simulink library "lib_AC_GFM"  (R2026a)
settings: Solver=VariableStepAuto
undefined symbols (not defined in the file): block_buses, block_idx, block_toM, buses_lf, fref, iC, invL, iR, iTf, op_GFM
libraries: simulink x4
(part 1 of 2)
settings Model: Creator=atomas  LastModifiedBy=atomas

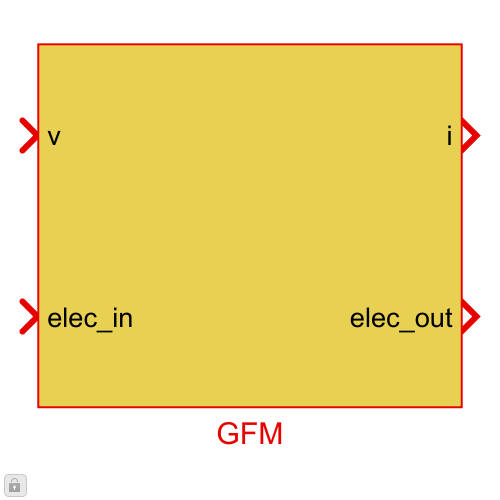
[thumbnail: Simulink's stored preview of the top-level diagram]
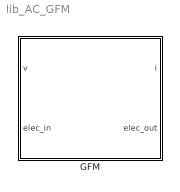
== system lib_AC_GFM ==
  GFM : Subsystem  mask(GFr){Pmax=Inf, Qmax=Inf, fb=50, dynamic_VCC=Static, Lf=0.01, Rf=0.001, Rcf=1000000, Cfi=0.1, Kint=1, Tint=0.1, Bint=1, Kext=1, Bext=1, Text=0.1, Fi=1, Tf=0.01, mp=0.01, mD=0, nq=0.01, VI_L=0.1, VI_R=0.01, WOF_Tf=0, L_out=0.1, R_out=0.01}
      mask prompts: Pmax "Active power limit (p.u.)"; Qmax "Reactive power limit (p.u.)"; fb "Base frequency (Hz)"; dynamic_VCC "Dynamic behavior"; Lf "Filter inductance (pu)"; Rf "Filter resistance (pu)"; Rcf "Parallel resistance to C (pu)"; Cfi "Filter capacitance (pu)"; Fi "Current feedfordward gain"; Tf "Low-pass filter time constant (s)"; mp "Droop coefficient mp (pu)"; mD "Droop coefficient mD (pu)"; nq "Droop coefficient nq (pu)"; VI_L "Inductance (pu)"; VI_R "Resistance (pu)"; WOF_Tf "WOF time constant (s)"; L_out "Output inductance (p.u.)"; R_out "Output resistance (p.u.)"
      mask help: Grid-forming converter. VCC are the voltage and current controllers. Dynamic behavior includes the PI controllers, decoupling, current feedfordward and LC output filter. Static behavior consists of setting the reference voltage directly in the output. PC is the power controller including the droop control and low-pass filters for the power measurements.
      mask init:
      | [block_buses, block_idx, block_toM, block_fref, vcc_mode] = mask_init_GFM(gcb, dynamic_VCC);
      mask Help: web('doc_GFr.html')
      mask TypeOptions dynamic_VCC: Dynamic with limitation | Dynamic | Static | Dynamic VC and static CC
      mask TypeOptions Tf: PC/Tf
      mask TypeOptions mp: PC/mp
      mask TypeOptions nq: PC/nq
      mask TypeOptions VI_L: VI/L
      mask TypeOptions VI_R: VI/R
      mask TypeOptions WOF_Tf: VI/Tf
      mask DialogControl Container8 Prompt: Parameters
      mask DialogControl VCC Prompt: VCC
      mask DialogControl PC Prompt: PC
      mask DialogControl VI Prompt: VI
      mask DialogControl Container9 Prompt: Others

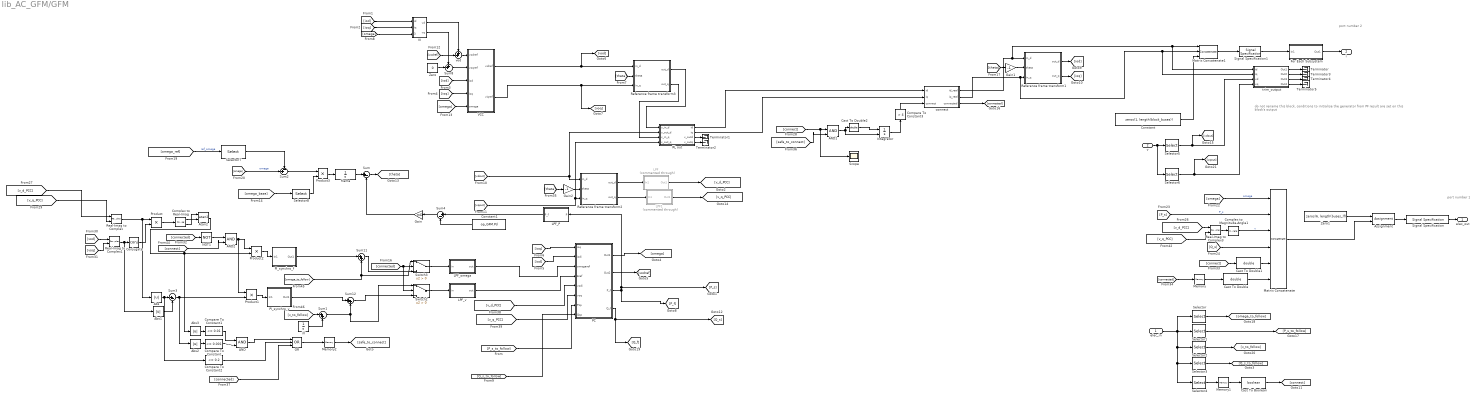
== system lib_AC_GFM/GFM ==
  note: port number 1
  note: do not rename this block, conditions to initialise the generator from PF result are set on this block's output
  note: port number 2
  elec_in : Inport
  v : Inport  Port=2
  AND : Logic  IconShape=distinctive  AllPortsSameDT=off  OutDataTypeStr=boolean
  AND1 : Logic  IconShape=distinctive  AllPortsSameDT=off  OutDataTypeStr=boolean
  AND2 : Logic  IconShape=distinctive  AllPortsSameDT=off  OutDataTypeStr=boolean
  Abs{,1..3} (4 alike) : Abs  ZeroCross=off  SaturateOnIntegerOverflow=off
  Assignment : Assignment  NumberOfDimensions=2  DiagnosticForDimensions=Warning  IndexOptions=Assign all,Index vector (dialog)  Indices=1,block_idx  OutputSizes=1,1
  Atan2 : Trigonometry  Operator=atan2
  Cast To Boolean : DataTypeConversion  OutDataTypeStr=boolean  SaturateOnIntegerOverflow=off  RndMeth=Floor
  Cast To Double : DataTypeConversion  OutDataTypeStr=double  SaturateOnIntegerOverflow=off  RndMeth=Floor
  Cast To Double1 : DataTypeConversion  OutDataTypeStr=double  SaturateOnIntegerOverflow=off  RndMeth=Floor
  Cast To Double2 : DataTypeConversion  OutDataTypeStr=double  SaturateOnIntegerOverflow=off  RndMeth=Floor
  Compare To Constant : simulink/Logic and Bit Operations/Compare To Constant  relop=<=  const=0.001  OutDataTypeStr=boolean  ZeroCross=off
  Compare To Constant1 : simulink/Logic and Bit Operations/Compare To Constant  relop=<=  const=0.01  OutDataTypeStr=boolean  ZeroCross=off
  Compare To Constant2 : simulink/Logic and Bit Operations/Compare To Constant  relop=<=  const=0.2  OutDataTypeStr=boolean  ZeroCross=off
  Compare To Constant3 : simulink/Logic and Bit Operations/Compare To Constant  relop=>  const=4  OutDataTypeStr=boolean  ZeroCross=off
  Complex to Magnitude-Angle1 : ComplexToMagnitudeAngle  Output=Magnitude
  Complex to Real-Imag : ComplexToRealImag
  Conjugate : Math  Operator=conj  SignedPower=on  RndMeth=Zero
  Constant : Constant  Value=zeros(1, length(block_buses))  VectorParams1D=off
  Constant1 : Constant  Value=op_GFM.Pd
  For Each Subsystem : Subsystem  TreatAsAtomicUnit=on
  Gain : Gain  Gain=mD
  Gain1 : Gain  Gain=-1
  Gain2 : Gain  Gain=-1
  Integrator : Integrator  ExternalReset=falling  InitialCondition=op_GFM.Integrator
  LPF : Subsystem  Commented=through
  LPF1 : Subsystem  Commented=through
  LPF_P : Subsystem
  LPF_omega : Subsystem
  LPF_v : Subsystem
  Matrix Concatenate : Concatenate  NumInputs=6  Mode=Multidimensional array
  Matrix Concatenate1 : Concatenate  NumInputs=3  Mode=Multidimensional array
  Memory : Memory  InitialCondition=1
  Memory1 : Memory  InitialCondition=1
  Memory2 : Memory  InitialCondition=1
  NOT1 : Logic  Operator=NOT  IconShape=distinctive  AllPortsSameDT=off  OutDataTypeStr=boolean
  OR : Logic  Operator=OR  Inputs=3  IconShape=distinctive  AllPortsSameDT=off  OutDataTypeStr=boolean
  PC : Subsystem  mask(PC_VCVSC){Tf=Tf, mp=mp, nq=nq}
      mask prompts: Tf "Low-pass filter time constant (s)"; mp "Droop coefficient mp"; nq "Droop coefficient nq"
      mask help: Power controller of a grid-forming converter, including the droop control and low-pass filters for the power measurements.
      mask init:
      | [iTf, use_Tf] = mask_init_opt_filter(Tf);
  PI_synchro_f : Subsystem
  PI_synchro_v : Subsystem
  Product : Product
  Product1 : Product  OutDataTypeStr=double
  Product2 : Product  OutDataTypeStr=double
  Product3 : Product
  RL out : Subsystem  Variant=on  mask{dynamic=Dynamic, R=R_out, L=L_out}
      mask prompts: dynamic "Dynamic behavior"; R "Series resistance (p.u.)"; L "Inductance (p.u.)"
      mask init:
      | [invL, omegab, rl_mode] = mask_init_RL(dynamic, L, 50);
      mask TypeOptions dynamic: Static | Dynamic | Static omega
  Real-Imag to Complex : RealImagToComplex
  Real-Imag to Complex1 : RealImagToComplex
  Real-Imag to Complex3 : RealImagToComplex
  Reference frame transform1 : Subsystem
  Reference frame transform2 : Subsystem
  Reference frame transform3 : Subsystem
  Scope : Scope
      settings: ActiveDisplayYMinimum=0.9  ActiveDisplayYMaximum=1.1
  Selector : Selector  NumberOfDimensions=2  InputPortWidth=3  IndexOptions=Index vector (dialog),Index vector (dialog)  Indices=1,block_idx  OutputSizes=1,1
  Selector1 : Selector  NumberOfDimensions=2  InputPortWidth=3  IndexOptions=Index vector (dialog),Index vector (dialog)  Indices=2,block_idx  OutputSizes=1,1
  Selector2 : Selector  NumberOfDimensions=2  InputPortWidth=3  IndexOptions=Index vector (dialog),Index vector (dialog)  Indices=3,block_idx  OutputSizes=1,1
  Selector3 : Selector  NumberOfDimensions=2  InputPortWidth=3  IndexOptions=Index vector (dialog),Index vector (dialog)  Indices=4,block_idx  OutputSizes=1,1
  Selector4 : Selector  NumberOfDimensions=2  InputPortWidth=3  IndexOptions=Index vector (dialog),Index vector (dialog)  Indices=5,block_idx  OutputSizes=1,1
  Selector5 : Selector  NumberOfDimensions=2  InputPortWidth=3  IndexOptions=Index vector (dialog),Index vector (dialog)  Indices=1,block_buses  OutputSizes=1,1
  Selector6 : Selector  NumberOfDimensions=2  InputPortWidth=3  IndexOptions=Index vector (dialog),Index vector (dialog)  Indices=2,block_buses  OutputSizes=1,1
  Selector7 : Selector  InputPortWidth=length(fref.ref_units)  IndexOptions=Index vector (dialog)  Indices=block_fref  OutputSizes=1
  Selector8 : Selector  InputPortWidth=length(fref.ref_units)  IndexOptions=Index vector (dialog)  Indices=block_fref  OutputSizes=1
  Signal Specification : SignalSpecification  Dimensions=[6 length(buses_lf)]
  Signal Specification1 : SignalSpecification  Dimensions=[3 length(block_buses)]
  Sum : Sum  Inputs=|+-
  Sum1 : Sum  Inputs=|++
  Sum11 : Sum  Inputs=|++
  Sum12 : Sum  Inputs=|++
  Sum2 : Sum  Inputs=-+|
  Sum3 : Sum  Inputs=|+-
  Sum4 : Sum  Inputs=|+-
  Sum8 : Sum  Inputs=++|
  Switch2 : Switch  Criteria=u2 > Threshold  SaturateOnIntegerOverflow=off  InputSameDT=off
  Switch3 : Switch  Criteria=u2 > Threshold  SaturateOnIntegerOverflow=off  InputSameDT=off
  Terminator{,1..5} (6 alike) : Terminator
  VCC : Subsystem  Variant=on
  VI : Subsystem  mask{L=VI_L, R=VI_R, Tf=WOF_Tf}
      mask prompts: L "Inductance (pu)"; R "Resistance (pu)"; Tf "WOF time constant (s)"
      mask init:
      | [iTf, use_Tf] = mask_init_opt_filter(Tf);
  Zero : Constant  Value=0  OutDataTypeStr=Inherit: Inherit via back propagation
  Zero1 : Constant  Value=zeros(6, length(buses_lf))  VectorParams1D=off  OutDataTypeStr=Inherit: Inherit via back propagation
  connect : Subsystem
  frame : Integrator  InitialCondition=op_GFM.frame  IgnoreLimit=on
  iV : Integrator  InitialCondition=op_GFM.iV
  trim_output : Subsystem
  vod : Sum  Inputs=++|
  elec_out : Outport
  i : Outport  Port=2
  wires:
  Sum8/1 -> VCC/2(voqref)
  vod/1 -> VCC/1(vodref)
  [omega] -> VI/3(omega)
  [ioq] -> VI/2(iq)
  [iod] -> VI/1(id)
  Gain2/1 -> Reference frame transform2/2(theta)
  [theta] -> Gain2/1
  connect/3(connected) -> [connected]
  [omega] -> Sum2/2  "omega"
  [omega_ref] -> Selector7/1  "ref_omega"
  RL out/1(id) -> connect/1(id)
  [theta] -> Gain1/1
  Gain1/1 -> Reference frame transform1/2(theta)
  [ioq] -> VCC/4(ioq)
  [iod] -> VCC/3(iod)
  Zero/1 -> Sum8/2
  [vodref] -> vod/2
  [omega] -> VCC/5(omega)
  [theta] -> Reference frame transform3/2(theta)
  PC/1(Out1) -> [omega]
  PC/2(Out2) -> [vodref]
  [iod] -> PC/2(iodi)
  [ioq] -> PC/1(ioq)
  Reference frame transform1/2(out_q) -> [ioq]
  Reference frame transform3/1(out_d) -> RL out/1(v_in_d)
  Reference frame transform3/2(out_q) -> RL out/3(v_in_q)
  RL out/2(iq) -> connect/2(iq)
  Reference frame transform1/1(out_d) -> [iod]
  VI/1(vd) -> vod/1
  VI/2(vq) -> Sum8/1
  connect/1(id_real) -> trim_output/1(id), Matrix Concatenate1/1, Reference frame transform1/1(in_d)
  connect/2(iq_real) -> trim_output/2(iq), Matrix Concatenate1/2, Reference frame transform1/3(in_q)
  RL out/3(v_outd) -> Terminator1/1
  RL out/4(v_outq) -> Terminator2/1
  Selector3/1 -> [Q_s_to_follow]
  Selector/1 -> [omega_to_follow]
  Selector2/1 -> [v_to_follow]
  [Q_s] -> Matrix Concatenate/4
  [P_s] -> Matrix Concatenate/2  "P_s"
  Complex to Magnitude-Angle1/1 -> Matrix Concatenate/3  "v"
  Matrix Concatenate/1 -> Assignment/2
  elec_in/1 -> Selector4/1, Selector3/1, Selector2/1, Selector1/1, Selector/1
  Assignment/1 -> Signal Specification/1
  [connect] -> Cast To Double1/1
  [connected] -> Memory/1
  Selector4/1 -> Memory1/1
  Cast To Double/1 -> Matrix Concatenate/6
  Cast To Double1/1 -> Matrix Concatenate/5
  Reference frame transform2/1(out_d) -> LPF/1(In1)
  Reference frame transform2/2(out_q) -> LPF1/1(In1)
  [v_d_PCC] -> Real-Imag to Complex/1
  [v_q_PCC] -> Real-Imag to Complex/2
  [vod] -> Real-Imag to Complex1/1
  [voq] -> Real-Imag to Complex1/2
  Real-Imag to Complex1/1 -> Abs1/1, Conjugate/1
  Real-Imag to Complex/1 -> Abs/1, Product/1
  Conjugate/1 -> Product/2
  Product/1 -> Complex to Real-Imag/1
  Complex to Real-Imag/2 -> Atan2/1
  Complex to Real-Imag/1 -> Atan2/2
  Abs/1 -> Compare To Constant2/1, Sum3/1
  Sum3/1 -> Abs2/1, Product1/2
  Product1/1 -> PI_synchro_v/1(In1)
  Product2/1 -> PI_synchro_f/1(In1)
  Atan2/1 -> Abs3/1, Product2/2
  Cast To Boolean/1 -> [connect]
  Abs1/1 -> Sum3/2
  Signal Specification/1 -> elec_out/1
  Abs2/1 -> Compare To Constant/1
  Compare To Constant/1 -> AND/2
  Abs3/1 -> Compare To Constant1/1
  Compare To Constant1/1 -> AND/1
  AND/1 -> OR/1
  OR/1 -> Memory2/1
  [connected] -> OR/3
  Memory2/1 -> [safe_to_connect]
  [vqout] -> Reference frame transform2/3(in_q), RL out/4(v_out_q)
  LPF/1(Out1) -> [v_d_PCC]
  LPF1/1(Out1) -> [v_q_PCC]
  [vdout] -> RL out/2(v_out_d), Reference frame transform2/1(in_d)
  Matrix Concatenate1/1 -> Signal Specification1/1
  Constant/1 -> Matrix Concatenate1/3
  For Each Subsystem/1(Out1) -> i/1
  Signal Specification1/1 -> For Each Subsystem/1(In1)
  [v_d_PCC] -> PC/5(vodi)
  [v_q_PCC] -> PC/6(voq)
  Real-Imag to Complex3/1 -> Complex to Magnitude-Angle1/1
  [v_q_PCC] -> Real-Imag to Complex3/2
  [v_d_PCC] -> Real-Imag to Complex3/1
  Zero1/1 -> Assignment/1
  trim_output/1(Out1) -> Terminator/1
  trim_output/2(Out2) -> Terminator3/1
  trim_output/3(Out3) -> Terminator4/1
  trim_output/4(Out4) -> Terminator5/1
  v/1 -> Selector6/1, Selector5/1
  Selector6/1 -> [vqout], trim_output/4(vq)
  Selector5/1 -> [vdout], trim_output/3(vd)
  Memory/1 -> Cast To Double/1
  Selector1/1 -> [P_s_to_follow]
  NOT1/1 -> AND2/1
  [connected] -> NOT1/1
  AND2/1 -> Product1/1, Product2/1
  [connect] -> Scope/1, AND1/1
  [safe_to_connect] -> AND1/2
  AND1/1 -> Integrator/2, Cast To Double2/1
  Cast To Double2/1 -> Integrator/1
  Memory1/1 -> Cast To Boolean/1
  VCC/1(vidref) -> [vod], Reference frame transform3/1(in_d)
  VCC/2(viqref) -> [voq], Reference frame transform3/3(in_q)
  Sum12/1 -> Switch2/3
  Sum1/1 -> Switch2/1, Sum12/2
  [omega_to_follow] -> Sum11/2, Switch3/1
  [connected] -> Switch2/2, Switch3/2
  Sum11/1 -> Switch3/3
  [P_s_to_follow] -> PC/7(Psp)
  [Q_s_to_follow] -> PC/8(Qsp)
  [v_to_follow] -> Sum1/1
  iV/1 -> Sum1/2
  [connect] -> AND2/2
  Switch3/1 -> LPF_omega/1(in)
  Switch2/1 -> LPF_v/1(in)
  PI_synchro_f/1(Out1) -> Sum11/1
  PI_synchro_v/1(Out1) -> Sum12/1
  LPF_v/1(out) -> PC/4(Eref)
  LPF_omega/1(out) -> PC/3(omegaref)
  Selector7/1 -> Sum2/1
  [omega_base] -> Selector8/1
  Product3/1 -> frame/1
  Selector8/1 -> Product3/2
  Sum2/1 -> Product3/1
  PC/4(Q_f) -> [Q_s], [Q_f]
  [omega] -> Matrix Concatenate/1  "omega"
  Integrator/1 -> Compare To Constant3/1
  Compare To Constant3/1 -> connect/3(connect)
  Compare To Constant2/1 -> OR/2
  frame/1 -> Sum/1
  Sum/1 -> [theta]
  PC/3(P_f) -> LPF_P/1(P), [P_s], [P_f]
  Sum4/1 -> Gain/1
  Constant1/1 -> Sum4/2
  LPF_P/1(P_f) -> Sum4/1
  Gain/1 -> Sum/2

== system lib_AC_GFM/GFM/For Each Subsystem ==
  In1 : Inport  Partition=on  PartitionDimension=1  PartitionWidth=1  PartitionOffset=0
  For Each : ForEach  DisableCoverage=on
  State-Space : StateSpace  A=[]  B=[]  C=[]  D=block_toM  InitialCondition=0  ParameterTunability=Optimized
  Transpose : Math  Operator=transpose
  Transpose1 : Math  Operator=transpose
  Out1 : Outport  ConcatenationDimension=1
  wires:
  In1/1 -> Transpose/1
  State-Space/1 -> Transpose1/1
  Transpose/1 -> State-Space/1
  Transpose1/1 -> Out1/1

== system lib_AC_GFM/GFM/LPF ==
  In1 : Inport
  Gain : Gain  Gain=1e2
  I : Integrator  InitialCondition=op_GFM.LPF_I
  Sum4 : Sum  Inputs=|+-
  Out1 : Outport
  wires:
  Gain/1 -> I/1
  Sum4/1 -> Gain/1
  In1/1 -> Sum4/1
  I/1 -> Out1/1, Sum4/2

== system lib_AC_GFM/GFM/LPF1 ==
  In1 : Inport
  Gain : Gain  Gain=1e2
  I : Integrator  InitialCondition=op_GFM.LPF1_I
  Sum4 : Sum  Inputs=|+-
  Out1 : Outport
  wires:
  I/1 -> Sum4/2, Out1/1
  In1/1 -> Sum4/1
  Sum4/1 -> Gain/1
  Gain/1 -> I/1

== system lib_AC_GFM/GFM/LPF_P ==
  P : Inport
  Gain : Gain  Gain=100
  I : Integrator  InitialCondition=op_GFM.LPF_P_I
  Sum4 : Sum  Inputs=|+-
  P_f : Outport
  wires:
  Gain/1 -> I/1
  Sum4/1 -> Gain/1
  P/1 -> Sum4/1
  I/1 -> P_f/1, Sum4/2

== system lib_AC_GFM/GFM/LPF_omega ==
  in : Inport
  Gain : Gain  Gain=100
  I : Integrator  InitialCondition=op_GFM.LPF_omega_I
  Sum4 : Sum  Inputs=|+-
  out : Outport
  wires:
  Gain/1 -> I/1
  Sum4/1 -> Gain/1
  in/1 -> Sum4/1
  I/1 -> Sum4/2, out/1

== system lib_AC_GFM/GFM/LPF_v ==
  in : Inport
  Gain : Gain  Gain=100
  I : Integrator  InitialCondition=op_GFM.LPF_v_I
  Sum4 : Sum  Inputs=|+-
  out : Outport
  wires:
  Gain/1 -> I/1
  Sum4/1 -> Gain/1
  in/1 -> Sum4/1
  I/1 -> Sum4/2, out/1

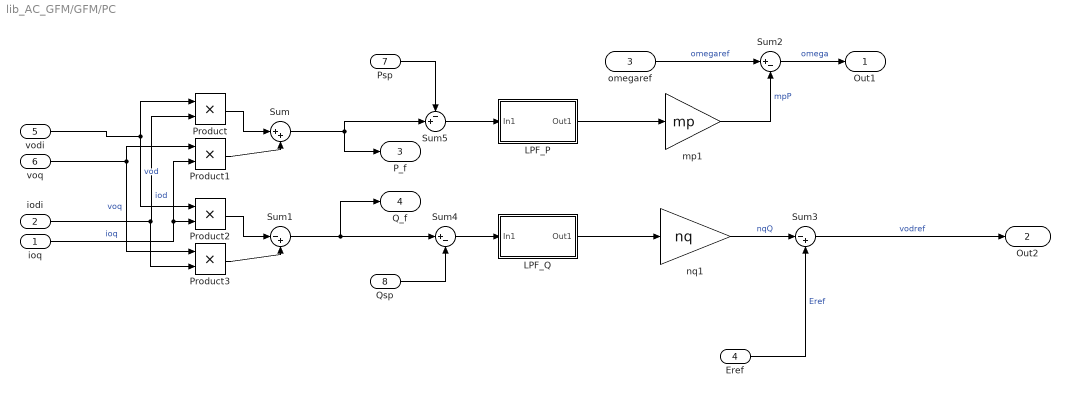
== system lib_AC_GFM/GFM/PC ==
  ioq : Inport
  iodi : Inport  Port=2
  omegaref : Inport  Port=3
  Eref : Inport  Port=4
  vodi : Inport  Port=5
  voq : Inport  Port=6
  Psp : Inport  Port=7
  Qsp : Inport  Port=8
  LPF_P : Subsystem  Variant=on
  LPF_Q : Subsystem  Variant=on
  Product{,1..3} (4 alike) : Product
  Sum : Sum  Inputs=|++
  Sum1 : Sum  Inputs=|-+
  Sum2 : Sum  Inputs=|+-
  Sum3 : Sum  Inputs=|-+
  Sum4 : Sum  Inputs=|+-
  Sum5 : Sum  Inputs=-+|
  mp1 : Gain  Gain=mp
  nq1 : Gain  Gain=nq
  Out1 : Outport
  Out2 : Outport  Port=2
  P_f : Outport  Port=3
  Q_f : Outport  Port=4
  wires:
  LPF_Q/1(Out1) -> nq1/1
  Sum4/1 -> LPF_Q/1(In1)
  LPF_P/1(Out1) -> mp1/1
  Sum5/1 -> LPF_P/1(In1)
  Sum2/1 -> Out1/1  "omega"
  vodi/1 -> Product2/1, Product/1  "vod"
  Product/1 -> Sum/1
  Product1/1 -> Sum/2
  Product2/1 -> Sum1/1
  Product3/1 -> Sum1/2
  nq1/1 -> Sum3/1  "nqQ"
  Eref/1 -> Sum3/2  "Eref"
  omegaref/1 -> Sum2/1  "omegaref"
  Sum/1 -> Sum5/2, P_f/1
  Sum1/1 -> Q_f/1, Sum4/1
  mp1/1 -> Sum2/2  "mpP"
  voq/1 -> Product1/1, Product3/1  "voq"
  iodi/1 -> Product3/2, Product/2  "iod"
  ioq/1 -> Product2/2, Product1/2  "ioq"
  Qsp/1 -> Sum4/2
  Sum3/1 -> Out2/1  "vodref"
  Psp/1 -> Sum5/1

== system lib_AC_GFM/GFM/PI_synchro_f ==
  In1 : Inport
  Gain : Gain  Gain=0.1
  Gain1 : Gain  Gain=0.2
  I : Integrator  InitialCondition=op_GFM.PI_synchro_f_I
  Sum10 : Sum  Inputs=|++
  Out1 : Outport
  wires:
  Sum10/1 -> Out1/1
  Gain/1 -> Sum10/1
  I/1 -> Sum10/2
  Gain1/1 -> I/1
  In1/1 -> Gain/1, Gain1/1

== system lib_AC_GFM/GFM/PI_synchro_v ==
  In1 : Inport
  Gain : Gain  Gain=0.1
  Gain1 : Gain  Gain=0.2
  Gain2 : Gain  Gain=5
  I : Integrator  InitialCondition=op_GFM.PI_synchro_v_I
  Sum10 : Sum  Inputs=|++
  Out1 : Outport
  wires:
  Gain1/1 -> I/1
  I/1 -> Sum10/2
  Gain/1 -> Sum10/1
  Sum10/1 -> Out1/1
  In1/1 -> Gain2/1
  Gain2/1 -> Gain/1, Gain1/1

== system lib_AC_GFM/GFM/RL out ==
  note: 1) Add Subsystem or Model blocks as valid variant choices.
      | 2) You cannot connect blocks at this level. At simulation, connectivity is automatically
      | determined, based on the active variant and port name matching.
  v_in_d : Inport
  v_out_d : Inport  Port=2
  v_in_q : Inport  Port=3
  v_out_q : Inport  Port=4
  dynamic : Subsystem  VariantControl=rl_mode == 1
  static : Subsystem  VariantControl=rl_mode == 2
  static_omega : Subsystem  VariantControl=(default)
  id : Outport
  iq : Outport  Port=2
  v_outd : Outport  Port=3
  v_outq : Outport  Port=4

== system lib_AC_GFM/GFM/Reference frame transform1 ==
  in_d : Inport
  theta : Inport  Port=2
  in_q : Inport  Port=3
  Complex to Real-Imag : ComplexToRealImag
  Cos : Trigonometry  SCDEnableBlockLinearizationSpecification=on  Operator=cos
  Product : Product
  Real-Imag to Complex : RealImagToComplex
  Real-Imag to Complex1 : RealImagToComplex
  Sin : Trigonometry  SCDEnableBlockLinearizationSpecification=on
  out_d : Outport
  out_q : Outport  Port=2
  wires:
  Complex to Real-Imag/2 -> out_q/1
  Real-Imag to Complex1/1 -> Product/1
  Real-Imag to Complex/1 -> Product/2
  Product/1 -> Complex to Real-Imag/1
  theta/1 -> Sin/1, Cos/1
  Cos/1 -> Real-Imag to Complex1/1
  Sin/1 -> Real-Imag to Complex1/2
  Complex to Real-Imag/1 -> out_d/1
  in_q/1 -> Real-Imag to Complex/2
  in_d/1 -> Real-Imag to Complex/1

== system lib_AC_GFM/GFM/Reference frame transform2 ==
  in_d : Inport
  theta : Inport  Port=2
  in_q : Inport  Port=3
  Complex to Real-Imag : ComplexToRealImag
  Cos : Trigonometry  SCDEnableBlockLinearizationSpecification=on  Operator=cos
  Product : Product
  Real-Imag to Complex : RealImagToComplex
  Real-Imag to Complex1 : RealImagToComplex
  Sin : Trigonometry  SCDEnableBlockLinearizationSpecification=on
  out_d : Outport
  out_q : Outport  Port=2
  wires:
  in_d/1 -> Real-Imag to Complex/1
  in_q/1 -> Real-Imag to Complex/2
  Complex to Real-Imag/1 -> out_d/1
  Sin/1 -> Real-Imag to Complex1/2
  Cos/1 -> Real-Imag to Complex1/1
  theta/1 -> Cos/1, Sin/1
  Product/1 -> Complex to Real-Imag/1
  Real-Imag to Complex/1 -> Product/2
  Real-Imag to Complex1/1 -> Product/1
  Complex to Real-Imag/2 -> out_q/1

== system lib_AC_GFM/GFM/Reference frame transform3 ==
  in_d : Inport
  theta : Inport  Port=2
  in_q : Inport  Port=3
  Complex to Real-Imag : ComplexToRealImag
  Cos : Trigonometry  SCDEnableBlockLinearizationSpecification=on  Operator=cos
  Product : Product
  Real-Imag to Complex : RealImagToComplex
  Real-Imag to Complex1 : RealImagToComplex
  Sin : Trigonometry  SCDEnableBlockLinearizationSpecification=on
  out_d : Outport
  out_q : Outport  Port=2
  wires:
  Complex to Real-Imag/2 -> out_q/1
  Real-Imag to Complex1/1 -> Product/1
  Real-Imag to Complex/1 -> Product/2
  Product/1 -> Complex to Real-Imag/1
  theta/1 -> Cos/1, Sin/1
  Cos/1 -> Real-Imag to Complex1/1
  Sin/1 -> Real-Imag to Complex1/2
  Complex to Real-Imag/1 -> out_d/1
  in_q/1 -> Real-Imag to Complex/2
  in_d/1 -> Real-Imag to Complex/1

== system lib_AC_GFM/GFM/VCC ==
  note: 1) Add Subsystem or Model blocks as valid variant choices.
      | 2) You cannot connect blocks at this level. At simulation, connectivity is automatically
      | determined, based on the active variant and port name matching.
  vodref : Inport
  voqref : Inport  Port=2
  iod : Inport  Port=3
  ioq : Inport  Port=4
  omega : Inport  Port=5
  dynamic : Subsystem  VariantControl=vcc_mode == 1
  dynamic_VC : Subsystem  VariantControl=vcc_mode == 3
  dynamic_limiting : Subsystem  VariantControl=vcc_mode == 2
  static : Subsystem  VariantControl=(default)
  vidref : Outport
  viqref : Outport  Port=2

== system lib_AC_GFM/GFM/VI ==
  id : Inport
  iq : Inport  Port=2
  omega : Inport  Port=3
  Gain : Gain  Gain=L
  Gain1 : Gain  Gain=R
  Gain2 : Gain  Gain=L
  Gain3 : Gain  Gain=R
  Product : Product
  Product1 : Product
  Sum : Sum  Inputs=-+|
  Sum1 : Sum  Inputs=|--
  WOF_d : Subsystem  Variant=on
  WOF_q : Subsystem  Variant=on
  vd : Outport
  vq : Outport  Port=2
  wires:
  WOF_q/1(Out1) -> Gain/1, Gain3/1
  iq/1 -> WOF_q/1(In1)
  WOF_d/1(Out1) -> Gain1/1, Gain2/1
  id/1 -> WOF_d/1(In1)
  Sum1/1 -> vq/1
  Sum/1 -> vd/1
  Gain3/1 -> Sum1/2
  Gain1/1 -> Sum/1
  Product1/1 -> Sum1/1
  Gain2/1 -> Product1/2
  Product/1 -> Sum/2
  omega/1 -> Product1/1, Product/2
  Gain/1 -> Product/1

== system lib_AC_GFM/GFM/connect ==
  id : Inport
  iq : Inport  Port=2
  connect : Inport  Port=3
  Switch : Switch  Criteria=u2 > Threshold  ZeroCross=off  SaturateOnIntegerOverflow=off  InputSameDT=off
  Switch1 : Switch  Criteria=u2 > Threshold  ZeroCross=off  SaturateOnIntegerOverflow=off  InputSameDT=off
  Zero1 : Constant  Value=0  VectorParams1D=off  OutDataTypeStr=Inherit: Inherit via back propagation
  Zero2 : Constant  Value=0  VectorParams1D=off  OutDataTypeStr=Inherit: Inherit via back propagation
  id_real : Outport
  iq_real : Outport  Port=2
  connected : Outport  Port=3  OutDataTypeStr=boolean
  wires:
  Switch/1 -> id_real/1
  Zero1/1 -> Switch/3
  id/1 -> Switch/1
  connect/1 -> connected/1, Switch1/2, Switch/2
  Switch1/1 -> iq_real/1
  iq/1 -> Switch1/1
  Zero2/1 -> Switch1/3

== system lib_AC_GFM/GFM/trim_output ==
  id : Inport
  iq : Inport  Port=2
  vd : Inport  Port=3
  vq : Inport  Port=4
  Out1 : Outport
  Out2 : Outport  Port=2
  Out3 : Outport  Port=3
  Out4 : Outport  Port=4
  wires:
  id/1 -> Out1/1
  vq/1 -> Out4/1
  vd/1 -> Out3/1
  iq/1 -> Out2/1

== system lib_AC_GFM/GFM/PC/LPF_P ==
  note: 1) Add Subsystem or Model blocks as valid variant choices.
      | 2) You cannot connect blocks at this level. At simulation, connectivity is automatically
      | determined, based on the active variant and port name matching.
  In1 : Inport
  Active : Subsystem  VariantControl=use_Tf == 1
  Bypass : Subsystem  VariantControl=(default)
  Out1 : Outport

== system lib_AC_GFM/GFM/PC/LPF_Q ==
  note: 1) Add Subsystem or Model blocks as valid variant choices.
      | 2) You cannot connect blocks at this level. At simulation, connectivity is automatically
      | determined, based on the active variant and port name matching.
  In1 : Inport
  Active : Subsystem  VariantControl=use_Tf == 1
  Bypass : Subsystem  VariantControl=(default)
  Out1 : Outport

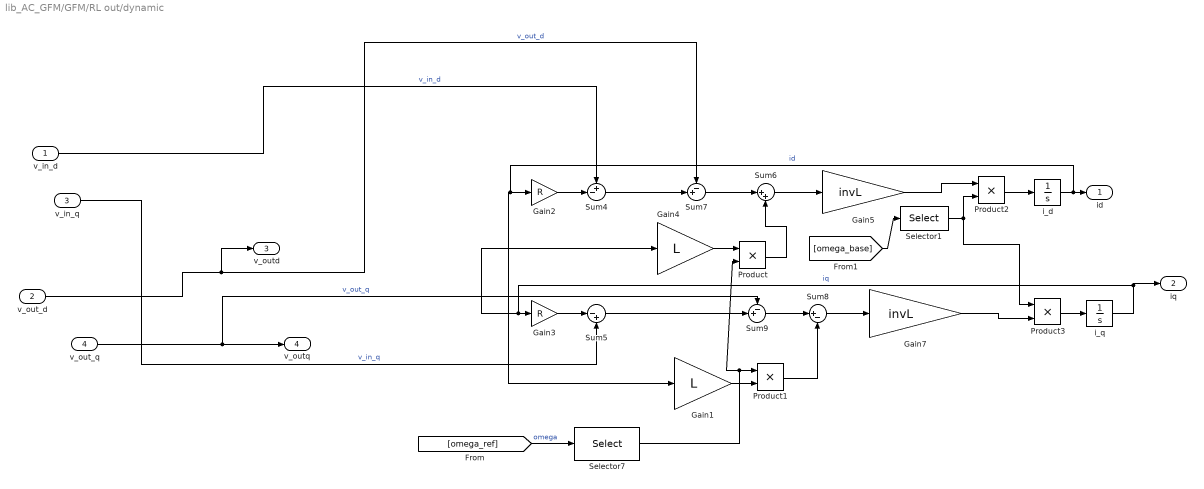
== system lib_AC_GFM/GFM/RL out/dynamic ==
  v_in_d : Inport
  v_out_d : Inport  Port=2
  v_in_q : Inport  Port=3
  v_out_q : Inport  Port=4
  Gain1 : Gain  Gain=L
  Gain2 : Gain  Gain=R
  Gain3 : Gain  Gain=R
  Gain4 : Gain  Gain=L
  Gain5 : Gain  Gain=invL
  Gain7 : Gain  Gain=invL
  Product{,1..3} (4 alike) : Product
  Selector1 : Selector  InputPortWidth=length(fref.ref_units)  IndexOptions=Index vector (dialog)  Indices=block_fref  OutputSizes=1
  Selector7 : Selector  InputPortWidth=length(fref.ref_units)  IndexOptions=Index vector (dialog)  Indices=block_fref  OutputSizes=1
  Sum4 : Sum  Inputs=+-|
  Sum5 : Sum  Inputs=|-+
  Sum6 : Sum  Inputs=|++
  Sum7 : Sum  Inputs=-+|
  Sum8 : Sum  Inputs=|+-
  Sum9 : Sum  Inputs=-+|
  i_d : Integrator  InitialCondition=op_GFM.RL_out_dynamic_i_d
  i_q : Integrator  InitialCondition=op_GFM.RL_out_dynamic_i_q
  id : Outport
  iq : Outport  Port=2
  v_outd : Outport  Port=3
  v_outq : Outport  Port=4
  wires:
  v_out_q/1 -> v_outq/1, Sum9/1  "v_out_q"
  v_out_d/1 -> v_outd/1, Sum7/1  "v_out_d"
  Sum9/1 -> Sum8/1
  Gain1/1 -> Product1/2
  i_q/1 -> iq/1, Gain4/1, Gain3/1  "iq"
  Sum5/1 -> Sum9/2
  Gain3/1 -> Sum5/1
  Sum7/1 -> Sum6/1
  Gain4/1 -> Product/1
  Product1/1 -> Sum8/2
  Sum4/1 -> Sum7/2
  Sum8/1 -> Gain7/1
  Product/1 -> Sum6/2
  [omega_ref] -> Selector7/1  "omega"
  Sum6/1 -> Gain5/1
  i_d/1 -> id/1, Gain1/1, Gain2/1  "id"
  Gain2/1 -> Sum4/2
  v_in_d/1 -> Sum4/1  "v_in_d"
  v_in_q/1 -> Sum5/2  "v_in_q"
  Selector7/1 -> Product/2, Product1/1
  Selector1/1 -> Product2/2, Product3/1
  [omega_base] -> Selector1/1
  Product3/1 -> i_q/1
  Gain7/1 -> Product3/2
  Gain5/1 -> Product2/1
  Product2/1 -> i_d/1

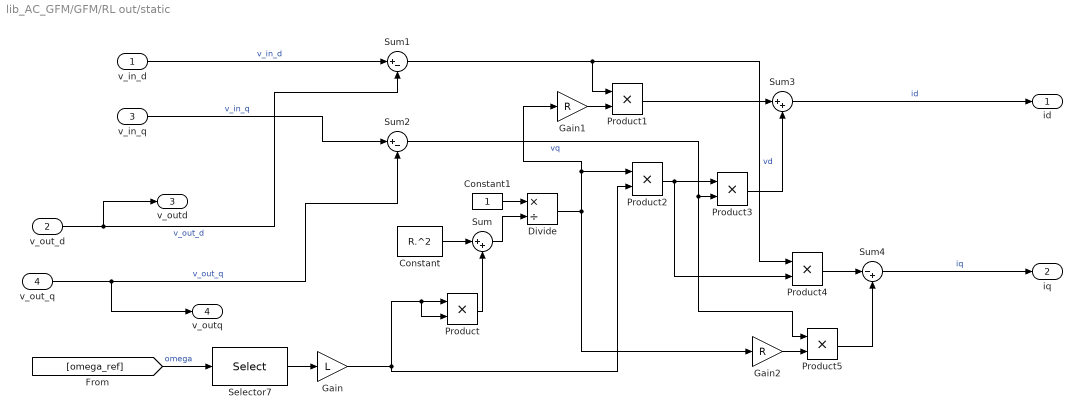
== system lib_AC_GFM/GFM/RL out/static ==
  v_in_d : Inport
  v_out_d : Inport  Port=2
  v_in_q : Inport  Port=3
  v_out_q : Inport  Port=4
  Constant : Constant  Value=R.^2
  Constant1 : Constant
  Divide : Product  Inputs=*/
  Gain : Gain  Gain=L
  Gain1 : Gain  Gain=R
  Gain2 : Gain  Gain=R
  Product{,1..5} (6 alike) : Product
  Selector7 : Selector  InputPortWidth=length(fref.ref_units)  IndexOptions=Index vector (dialog)  Indices=block_fref  OutputSizes=1
  Sum : Sum  Inputs=|++
  Sum1 : Sum  Inputs=|+-
  Sum2 : Sum  Inputs=|+-
  Sum3 : Sum  Inputs=|++
  Sum4 : Sum  Inputs=|-+
  id : Outport
  iq : Outport  Port=2
  v_outd : Outport  Port=3
  v_outq : Outport  Port=4
  wires:
  v_in_d/1 -> Sum1/1  "v_in_d"
  v_out_q/1 -> v_outq/1, Sum2/2  "v_out_q"
  Sum4/1 -> iq/1  "iq"
  Sum3/1 -> id/1  "id"
  Gain1/1 -> Product1/2
  Product2/1 -> Product4/2, Product3/1
  Product4/1 -> Sum4/1
  Divide/1 -> Gain2/1, Gain1/1, Product2/1
  Sum1/1 -> Product1/1, Product4/1  "vd"
  Product3/1 -> Sum3/2
  Constant1/1 -> Divide/1
  Gain/1 -> Product/2, Product/1, Product2/2
  Sum2/1 -> Product5/1, Product3/2  "vq"
  Constant/1 -> Sum/1
  Product5/1 -> Sum4/2
  Product1/1 -> Sum3/1
  Product/1 -> Sum/2
  Gain2/1 -> Product5/2
  Sum/1 -> Divide/2
  v_out_d/1 -> v_outd/1, Sum1/2  "v_out_d"
  v_in_q/1 -> Sum2/1  "v_in_q"
  [omega_ref] -> Selector7/1  "omega"
  Selector7/1 -> Gain/1

== system lib_AC_GFM/GFM/RL out/static_omega ==
  v_in_d : Inport
  v_out_d : Inport  Port=2
  v_in_q : Inport  Port=3
  v_out_q : Inport  Port=4
  Gain : Gain  Gain=1./(R.^2+L.^2)
  Gain2 : Gain  Gain=1./(R.^2+L.^2)
  Gain3 : Gain  Gain=R
  Gain4 : Gain  Gain=L
  Gain5 : Gain  Gain=L
  Gain6 : Gain  Gain=R
  Sum : Sum  Inputs=|++
  Sum1 : Sum  Inputs=|+-
  Sum2 : Sum  Inputs=|+-
  Sum3 : Sum  Inputs=|-+
  id : Outport
  iq : Outport  Port=2
  v_outd : Outport  Port=3
  v_outq : Outport  Port=4
  wires:
  v_in_q/1 -> Sum2/1  "v_in_q"
  v_in_d/1 -> Sum1/1  "v_in_d"
  v_out_q/1 -> v_outq/1, Sum2/2  "v_out_q"
  v_out_d/1 -> v_outd/1, Sum1/2  "v_out_d"
  Sum1/1 -> Gain/1  "vd"
  Sum2/1 -> Gain2/1  "vq"
  Gain/1 -> Gain5/1, Gain3/1
  Gain3/1 -> Sum/1
  Gain4/1 -> Sum/2
  Gain2/1 -> Gain6/1, Gain4/1
  Sum/1 -> id/1
  Gain5/1 -> Sum3/1
  Sum3/1 -> iq/1
  Gain6/1 -> Sum3/2

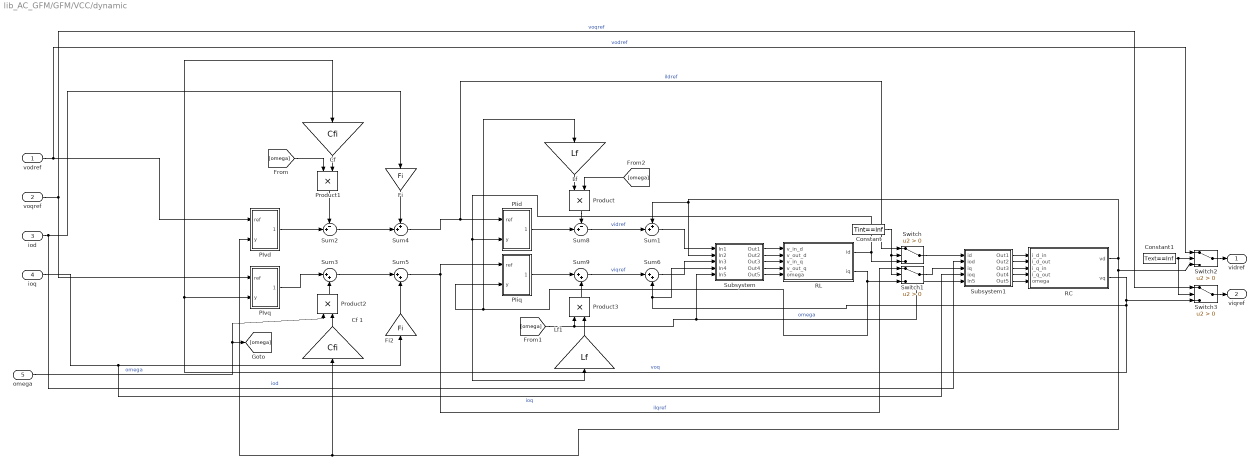
== system lib_AC_GFM/GFM/VCC/dynamic ==
  vodref : Inport
  voqref : Inport  Port=2
  iod : Inport  Port=3
  ioq : Inport  Port=4
  omega : Inport  Port=5
  Cf : Gain  Gain=Cfi
  Cf 1 : Gain  Gain=Cfi
  Constant : Constant  Value=Tint==Inf  VectorParams1D=off
  Constant1 : Constant  Value=Text==Inf  VectorParams1D=off
  Fi : Gain  Gain=Fi
  Fi2 : Gain  Gain=Fi
  "Lf " : Gain  Gain=Lf
  Lf1 : Gain  Gain=Lf
  PIid : Subsystem
  PIiq : Subsystem
  PIvd : Subsystem
  PIvq : Subsystem
  Product{,1..3} (4 alike) : Product
  RC : Subsystem  Variant=on  mask{dynamic=Dynamic, R=Rcf, C=Cfi}
      mask prompts: dynamic "Dynamic behavior"; R "Parallel resistance (p.u.)"; C "Capacitance (p.u.)"
      mask init:
      | [iC, iR, omegab, rc_mode] = mask_init_RC(dynamic, R, C, 50);
      mask TypeOptions dynamic: Dynamic | Static | Static omega
  RL : Subsystem  Variant=on  mask(Line){dynamic=Dynamic, R=Rf, L=Lf}
      mask prompts: dynamic "Dynamic behavior"; R "Series resistance (p.u.)"; L "Inductance (p.u.)"
      mask init:
      | [invL, omegab, rl_mode] = mask_init_RL(dynamic, L, 50);
      mask Help: web('Documentation/RL.html')
      mask TypeOptions dynamic: Static | Dynamic | Static omega
  Subsystem : Subsystem
  Subsystem1 : Subsystem
  Sum1 : Sum  Inputs=++|
  Sum2 : Sum  Inputs=-+|
  Sum{3,5..6,9} (4 alike) : Sum  Inputs=|++
  Sum4 : Sum  Inputs=++|
  Sum8 : Sum  Inputs=-+|
  Switch{,1..3} (4 alike) : Switch  Criteria=u2 > Threshold  SaturateOnIntegerOverflow=off  InputSameDT=off
  vidref : Outport
  viqref : Outport  Port=2
  wires:
  Sum5/1 -> Switch1/1, PIiq/1(ref)  "ilqref"
  Product/1 -> Sum8/1
  vodref/1 -> Switch2/1, PIvd/1(ref)  "vodref"
  RC/2(vq) -> PIvq/2(y), Cf/1, Subsystem/4(In4), Sum6/2, Switch3/3  "voq"
  [omega] -> Product/2
  Lf1/1 -> Product3/2
  Fi/1 -> Sum4/1
  voqref/1 -> Switch3/1, PIvq/1(ref)  "voqref"
  Product3/1 -> Sum9/2
  Product2/1 -> Sum3/2
  Cf 1/1 -> Product2/2
  Cf/1 -> Product1/2
  Sum4/1 -> PIid/1(ref), Switch/1  "ildref"
  Product1/1 -> Sum2/1
  iod/1 -> Subsystem1/2(iod), Fi/1  "iod"
  Sum2/1 -> Sum4/2
  "Lf "/1 -> Product/1
  Sum3/1 -> Sum5/1
  [omega] -> Subsystem1/5(In5), Subsystem/5(In5), Product3/1  "omega"
  ioq/1 -> Subsystem1/4(ioq), Fi2/1  "ioq"
  Fi2/1 -> Sum5/2
  PIvd/1(Out1) -> Sum2/2
  PIvq/1(Out1) -> Sum3/1
  PIid/1(Out1) -> Sum8/2
  PIiq/1(Out1) -> Sum9/1
  omega/1 -> Product2/1, [omega]  "omega"
  [omega] -> Product1/1
  RC/1(vd) -> Subsystem/2(In2), Sum1/1, Switch2/3, PIvd/2(y), Cf 1/1
  RL/1(id) -> Switch/3, Lf1/1, PIid/2(y)
  RL/2(iq) -> Switch1/3, PIiq/2(y), "Lf "/1
  Sum8/1 -> Sum1/2  "vidref"
  Sum9/1 -> Sum6/1  "viqref"
  Sum1/1 -> Subsystem/1(In1)
  Sum6/1 -> Subsystem/3(In3)
  Subsystem/1(Out1) -> RL/1(v_in_d)
  Subsystem/2(Out2) -> RL/2(v_out_d)
  Subsystem/3(Out3) -> RL/3(v_in_q)
  Subsystem/4(Out4) -> RL/4(v_out_q)
  Subsystem/5(Out5) -> RL/5(omega)
  Subsystem1/1(Out1) -> RC/1(i_d_in)
  Subsystem1/2(Out2) -> RC/2(i_d_out)
  Subsystem1/3(Out3) -> RC/3(i_q_in)
  Subsystem1/4(Out4) -> RC/4(i_q_out)
  Subsystem1/5(Out5) -> RC/5(omega)
  Switch/1 -> Subsystem1/1(id)
  Switch1/1 -> Subsystem1/3(iq)
  Constant/1 -> Switch1/2, Switch/2
  Switch2/1 -> vidref/1
  Constant1/1 -> Switch3/2, Switch2/2
  Switch3/1 -> viqref/1

== system lib_AC_GFM/GFM/VCC/dynamic_VC ==
  vodref : Inport
  voqref : Inport  Port=2
  iod : Inport  Port=3
  ioq : Inport  Port=4
  omega : Inport  Port=5
  Cf : Gain  Gain=Cfi
  Cf 1 : Gain  Gain=Cfi
  Fi : Gain  Gain=Fi
  Fi2 : Gain  Gain=Fi
  Product1 : Product
  Product2 : Product
  RC : Subsystem  Variant=on  mask{dynamic=Dynamic, R=Rcf, C=Cfi}
      mask prompts: dynamic "Dynamic behavior"; R "Parallel resistance (p.u.)"; C "Capacitance (p.u.)"
      mask init:
      | [iC, iR, omegab, rc_mode] = mask_init_RC(dynamic, R, C, 50);
      mask TypeOptions dynamic: Dynamic | Static | Static omega
  Subsystem : Subsystem
  Subsystem1 : Subsystem
  Sum2 : Sum  Inputs=-+|
  Sum3 : Sum  Inputs=|++
  Sum4 : Sum  Inputs=++|
  Sum5 : Sum  Inputs=|++
  vidref : Outport
  viqref : Outport  Port=2
  wires:
  [omega] -> Product1/1
  omega/1 -> RC/5(omega), Product2/1, [omega]  "omega"
  Subsystem1/1(Out1) -> Sum3/1
  Subsystem/1(Out1) -> Sum2/2
  Fi2/1 -> Sum5/2
  ioq/1 -> RC/4(i_q_out), Fi2/1  "ioq"
  Sum3/1 -> Sum5/1
  Sum2/1 -> Sum4/2
  iod/1 -> RC/2(i_d_out), Fi/1  "iod"
  Product1/1 -> Sum2/1
  Cf/1 -> Product1/2
  Cf 1/1 -> Product2/2
  Product2/1 -> Sum3/2
  voqref/1 -> Subsystem1/1(ref)  "voqref"
  Fi/1 -> Sum4/1
  RC/2(vq) -> viqref/1, Cf/1, Subsystem1/2(y)
  vodref/1 -> Subsystem/1(ref)  "vodref"
  RC/1(vd) -> vidref/1, Cf 1/1, Subsystem/2(y)
  Sum4/1 -> RC/1(i_d_in)
  Sum5/1 -> RC/3(i_q_in)

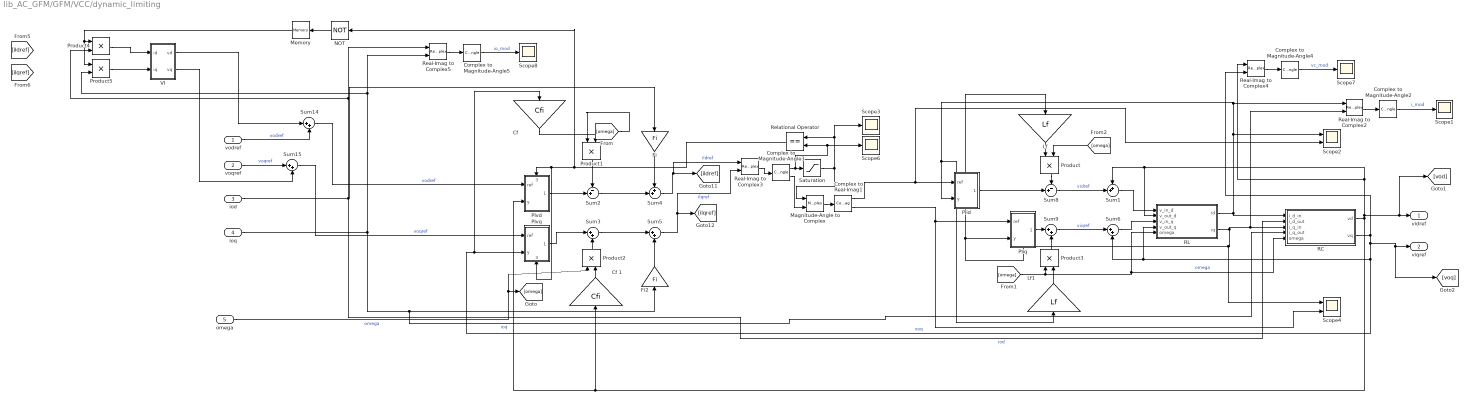
== system lib_AC_GFM/GFM/VCC/dynamic_limiting ==
  vodref : Inport
  voqref : Inport  Port=2
  iod : Inport  Port=3
  ioq : Inport  Port=4
  omega : Inport  Port=5
  Cf : Gain  Gain=Cfi
  Cf 1 : Gain  Gain=Cfi
  Complex to Magnitude-Angle2 : ComplexToMagnitudeAngle  Output=Magnitude
  Complex to Magnitude-Angle3 : ComplexToMagnitudeAngle
  Complex to Magnitude-Angle4 : ComplexToMagnitudeAngle  Output=Magnitude
  Complex to Magnitude-Angle5 : ComplexToMagnitudeAngle  Output=Magnitude
  Complex to Real-Imag1 : ComplexToRealImag
  Fi : Gain  Gain=Fi
  Fi2 : Gain  Gain=Fi
  "Lf " : Gain  Gain=Lf
  Lf1 : Gain  Gain=Lf
  Magnitude-Angle to Complex : MagnitudeAngleToComplex
  Memory : Memory
  NOT : Logic  Operator=NOT  IconShape=distinctive  AllPortsSameDT=off  OutDataTypeStr=boolean
  PIid : Subsystem
  PIiq : Subsystem
  PIvd : Subsystem
      settings: PortSchema="{\"entries\":[{\"content\":{\"sides\":[{\"content\":{\"connectorIds\":[\"In1\",\"In2\"]},\"type\":\"ConnectorPlacement.EquallySpacedRectSide\",\"uuid\":\"218efe14-094c-4cdd-8e62-ef6089c75bbd\"},{\"content\":{\"connectorIds\":[\"Out1\"],\"side\":\"RIGHT\"},\"type\":\"ConnectorPlacement.EquallySpacedRectSide\",\"uuid\":\"287e2a8a-062a-4519-a86c-f141c6982dac\"},{\"content\":{\"connectorIds\":[\"In3\"],\"side\":\"TOP\"},\"type\":\"ConnectorPlacement.EquallySpacedRectSide\",\"uuid\":\"e88fce21-908c-492a-b265-04b05ce94be8\"}]},\"type\":\"ConnectorPlacement.EquallySpacedConnector\",\"uuid\":\"5c149457-da6d-4223-b1cb-56365173b759\"}],\"packageUris\":[\"http://schema.mathworks.com/mf0/Connector/R2020b\"],\"version\":\"1.0\"}"
  PIvq : Subsystem
      settings: PortSchema="{\"entries\":[{\"content\":{\"sides\":[{\"content\":{\"connectorIds\":[\"In1\",\"In2\"]},\"type\":\"ConnectorPlacement.EquallySpacedRectSide\",\"uuid\":\"218efe14-094c-4cdd-8e62-ef6089c75bbd\"},{\"content\":{\"connectorIds\":[\"Out1\"],\"side\":\"RIGHT\"},\"type\":\"ConnectorPlacement.EquallySpacedRectSide\",\"uuid\":\"287e2a8a-062a-4519-a86c-f141c6982dac\"},{\"content\":{\"connectorIds\":[],\"side\":\"TOP\"},\"type\":\"ConnectorPlacement.EquallySpacedRectSide\",\"uuid\":\"e88fce21-908c-492a-b265-04b05ce94be8\"},{\"content\":{\"connectorIds\":[\"In3\"],\"side\":\"BOTTOM\"},\"type\":\"ConnectorPlacement.EquallySpacedRectSide\",\"uuid\":\"db964aea-37c6-4226-90b6-d177a6d2ab38\"}]},\"type\":\"ConnectorPlacement.EquallySpacedConnector\",\"uuid\":\"5c149457-da6d-4223-b1cb-56365173b759\"}],\"packageUris\":[\"http://schema.mathworks.com/mf0/Connector/R2020b\"],\"version\":\"1.0\"}"
  Product{,1..5} (6 alike) : Product
  RC : Subsystem  Variant=on  mask{dynamic=Dynamic, R=Rcf, C=Cfi}
      mask prompts: dynamic "Dynamic behavior"; R "Parallel resistance (p.u.)"; C "Capacitance (p.u.)"
      mask init:
      | [iC, iR, omegab, rc_mode] = mask_init_RC(dynamic, R, C, 50);
      mask TypeOptions dynamic: Dynamic | Static | Static omega
  RL : Subsystem  Variant=on  mask(Line){dynamic=Dynamic, R=Rf, L=Lf}
      mask prompts: dynamic "Dynamic behavior"; R "Series resistance (p.u.)"; L "Inductance (p.u.)"
      mask init:
      | [invL, omegab, rl_mode] = mask_init_RL(dynamic, L, 50);
      mask Help: web('Documentation/RL.html')
      mask TypeOptions dynamic: Static | Dynamic | Static omega
  Real-Imag to Complex{2..5} (4 alike) : RealImagToComplex
  Relational Operator : RelationalOperator  Operator===  OutDataTypeStr=boolean  RndMeth=Simplest  InputSameDT=off
  Saturation : Saturate  UpperLimit=0.1  LowerLimit=0
  Scope{1,3,6..8} (5 alike) : Scope
      Scope1 settings: ActiveDisplayYMinimum=-0.06728  ActiveDisplayYMaximum=0.79818  DataLoggingVariableName=ScopeData2
      Scope3 settings: ActiveDisplayYMinimum=0.01769  ActiveDisplayYMaximum=0.10915
      Scope6 settings: ActiveDisplayYMinimum=0.03196  ActiveDisplayYMaximum=0.13112  DataLoggingVariableName=ScopeData2
      Scope7 settings: ActiveDisplayYMinimum=0.86043  ActiveDisplayYMaximum=1.1554  DataLoggingVariableName=ScopeData3
      Scope8 settings: ActiveDisplayYMinimum=0.0318  ActiveDisplayYMaximum=0.12782  DataLoggingVariableName=ScopeData4
  Scope2 : Scope  NumInputPorts=2
      settings: ActiveDisplayYMinimum=-0.10019  ActiveDisplayYMaximum=0.20176
  Scope4 : Scope  NumInputPorts=2
      settings: ActiveDisplayYMinimum=-0.04364  ActiveDisplayYMaximum=0.0791  DataLoggingVariableName=ScopeData3
  Sum1 : Sum  Inputs=++|
  Sum{3,5..6,9,14..15} (6 alike) : Sum  Inputs=|++
  Sum2 : Sum  Inputs=-+|
  Sum4 : Sum  Inputs=++|
  Sum8 : Sum  Inputs=-+|
  VI : Subsystem  mask{L=0.5, R=0.1, Tf=0}
      mask prompts: L "Inductance (pu)"; R "Resistance (pu)"; Tf "WOF time constant (s)"
      mask init:
      | [iTf, use_Tf] = mask_init_opt_filter(Tf);
  vidref : Outport
  viqref : Outport  Port=2
  wires:
  Product/1 -> Sum8/1
  Sum14/1 -> PIvd/1(ref)  "vodref"
  RC/2(vq) -> [voq], viqref/1, RL/4(v_out_q), Sum6/2, PIvq/2(y), Cf/1, Real-Imag to Complex4/2  "voq"
  [omega] -> Product/2
  Lf1/1 -> Product3/2
  Fi/1 -> Sum4/1
  Sum15/1 -> PIvq/1(ref)  "voqref"
  Product3/1 -> Sum9/2
  Product2/1 -> Sum3/2
  Cf 1/1 -> Product2/2
  Cf/1 -> Product1/2
  Product1/1 -> Sum2/1
  iod/1 -> RC/2(i_d_out), Real-Imag to Complex5/1, Product4/2, Fi/1  "iod"
  Sum2/1 -> Sum4/2
  "Lf "/1 -> Product/1
  Sum3/1 -> Sum5/1
  [omega] -> RC/5(omega), RL/5(omega), Product3/1  "omega"
  ioq/1 -> RC/4(i_q_out), Fi2/1, Real-Imag to Complex5/2, Product5/2  "ioq"
  Fi2/1 -> Sum5/2
  PIvd/1(Out1) -> Sum2/2
  PIvq/1(Out1) -> Sum3/1
  PIid/1(Out1) -> Sum8/2
  PIiq/1(Out1) -> Sum9/1
  omega/1 -> Product2/1, [omega]  "omega"
  [omega] -> Product1/1
  RL/1(id) -> RC/1(i_d_in), Scope2/1, Real-Imag to Complex2/1, PIid/2(y), Lf1/1
  RL/2(iq) -> Scope4/1, PIiq/2(y), "Lf "/1, Real-Imag to Complex2/2, RC/3(i_q_in)
  Sum8/1 -> Sum1/2  "vidref"
  Sum9/1 -> Sum6/1  "viqref"
  Sum1/1 -> RL/1(v_in_d)
  Sum6/1 -> RL/3(v_in_q)
  Sum4/1 -> Real-Imag to Complex3/1, [ildref]  "ildref"
  Sum5/1 -> Real-Imag to Complex3/2, [ilqref]  "ilqref"
  RC/1(vd) -> Real-Imag to Complex4/1, RL/2(v_out_d), Sum1/1, [vod], vidref/1, PIvd/2(y), Cf 1/1
  Complex to Real-Imag1/2 -> Scope4/2, PIiq/1(ref)
  Real-Imag to Complex2/1 -> Complex to Magnitude-Angle2/1
  Complex to Magnitude-Angle2/1 -> Scope1/1  "i_mod"
  Complex to Real-Imag1/1 -> Scope2/2, PIid/1(ref)
  Real-Imag to Complex3/1 -> Complex to Magnitude-Angle3/1
  Saturation/1 -> Magnitude-Angle to Complex/1, Scope3/1, Relational Operator/1
  Relational Operator/1 -> PIvd/3(anti_windup), PIvq/3(anti_windup), NOT/1
  Complex to Magnitude-Angle3/1 -> Scope6/1, Relational Operator/2, Saturation/1
  Magnitude-Angle to Complex/1 -> Complex to Real-Imag1/1
  Complex to Magnitude-Angle3/2 -> Magnitude-Angle to Complex/2
  Complex to Magnitude-Angle4/1 -> Scope7/1  "vc_mod"
  Real-Imag to Complex4/1 -> Complex to Magnitude-Angle4/1
  Real-Imag to Complex5/1 -> Complex to Magnitude-Angle5/1
  Complex to Magnitude-Angle5/1 -> Scope8/1  "io_mod"
  vodref/1 -> Sum14/2  "vodref"
  voqref/1 -> Sum15/1  "voqref"
  NOT/1 -> Memory/1
  VI/1(vd) -> Sum14/1
  VI/2(vq) -> Sum15/2
  Memory/1 -> Product5/1, Product4/1
  Product4/1 -> VI/1(id)
  Product5/1 -> VI/2(iq)

== system lib_AC_GFM/GFM/VCC/static ==
  vodref : Inport
  voqref : Inport  Port=2
  iod : Inport  Port=3
  ioq : Inport  Port=4
  omega : Inport  Port=5
  Terminator : Terminator
  Terminator1 : Terminator
  Terminator2 : Terminator
  vidref : Outport
  viqref : Outport  Port=2
  wires:
  voqref/1 -> viqref/1  "voqref"
  vodref/1 -> vidref/1  "vodref"
  iod/1 -> Terminator/1  "iod"
  ioq/1 -> Terminator1/1  "ioq"
  omega/1 -> Terminator2/1  "ioq"

== system lib_AC_GFM/GFM/VI/WOF_d ==
  note: 1) Add Subsystem or Model blocks as valid variant choices.
      | 2) You cannot connect blocks at this level. At simulation, connectivity is automatically
      | determined, based on the active variant and port name matching.
  In1 : Inport
  Active : Subsystem  VariantControl=use_Tf == 1
  Bypass : Subsystem  VariantControl=(default)
  Out1 : Outport

== system lib_AC_GFM/GFM/VI/WOF_q ==
  note: 1) Add Subsystem or Model blocks as valid variant choices.
      | 2) You cannot connect blocks at this level. At simulation, connectivity is automatically
      | determined, based on the active variant and port name matching.
  In1 : Inport
  Active : Subsystem  VariantControl=use_Tf == 1
  Bypass : Subsystem  VariantControl=(default)
  Out1 : Outport

== system lib_AC_GFM/GFM/PC/LPF_P/Active ==
  In1 : Inport
  Impl : Subsystem
  Out1 : Outport
  wires:
  Impl/1(P_f) -> Out1/1
  In1/1 -> Impl/1(P)

== system lib_AC_GFM/GFM/PC/LPF_P/Bypass ==
  In1 : Inport
  Out1 : Outport
  wires:
  In1/1 -> Out1/1

== system lib_AC_GFM/GFM/PC/LPF_Q/Active ==
  In1 : Inport
  Impl : Subsystem
  Out1 : Outport
  wires:
  Impl/1(Q_f) -> Out1/1
  In1/1 -> Impl/1(Q)

== system lib_AC_GFM/GFM/PC/LPF_Q/Bypass ==
  In1 : Inport
  Out1 : Outport
  wires:
  In1/1 -> Out1/1

== system lib_AC_GFM/GFM/VCC/dynamic/PIid ==
  ref : Inport
  y : Inport  Port=2
  Gain : Gain  Gain=Bint
  Gain1 : Gain  Gain=1./Tint
  Gain2 : Gain  Gain=Kint
  I : Integrator  InitialCondition=op_GFM.VCC_dynamic_PIid_I
  Sum : Sum  Inputs=++|
  Sum1 : Sum  Inputs=|+-
  Sum6 : Sum  Inputs=|+-
  Out1 : Outport
  wires:
  y/1 -> Sum1/2, Sum6/2
  ref/1 -> Gain/1, Sum6/1
  Gain/1 -> Sum1/1
  Sum/1 -> Gain2/1
  Sum1/1 -> Sum/1
  Sum6/1 -> Gain1/1
  Gain1/1 -> I/1
  I/1 -> Sum/2
  Gain2/1 -> Out1/1

== system lib_AC_GFM/GFM/VCC/dynamic/PIiq ==
  ref : Inport
  y : Inport  Port=2
  Gain : Gain  Gain=Bint
  Gain1 : Gain  Gain=1./Tint
  Gain2 : Gain  Gain=Kint
  I : Integrator  InitialCondition=op_GFM.VCC_dynamic_PIiq_I
  Sum : Sum  Inputs=++|
  Sum1 : Sum  Inputs=|+-
  Sum6 : Sum  Inputs=|+-
  Out1 : Outport
  wires:
  Gain2/1 -> Out1/1
  I/1 -> Sum/2
  Gain1/1 -> I/1
  Sum6/1 -> Gain1/1
  Sum1/1 -> Sum/1
  Sum/1 -> Gain2/1
  Gain/1 -> Sum1/1
  ref/1 -> Sum6/1, Gain/1
  y/1 -> Sum6/2, Sum1/2

== system lib_AC_GFM/GFM/VCC/dynamic/PIvd ==
  ref : Inport
  y : Inport  Port=2
  Gain : Gain  Gain=Bext
  Gain1 : Gain  Gain=1./Text
  Gain2 : Gain  Gain=Kext
  I : Integrator  InitialCondition=op_GFM.VCC_dynamic_PIvd_I
  Sum : Sum  Inputs=++|
  Sum1 : Sum  Inputs=|+-
  Sum6 : Sum  Inputs=|+-
  Out1 : Outport
  wires:
  y/1 -> Sum1/2, Sum6/2
  ref/1 -> Gain/1, Sum6/1
  Gain/1 -> Sum1/1
  Sum/1 -> Gain2/1
  Sum1/1 -> Sum/1
  Sum6/1 -> Gain1/1
  Gain1/1 -> I/1
  I/1 -> Sum/2
  Gain2/1 -> Out1/1

== system lib_AC_GFM/GFM/VCC/dynamic/PIvq ==
  ref : Inport
  y : Inport  Port=2
  Gain : Gain  Gain=Bext
  Gain1 : Gain  Gain=1./Text
  Gain2 : Gain  Gain=Kext
  I : Integrator  InitialCondition=op_GFM.VCC_dynamic_PIvq_I
  Sum : Sum  Inputs=++|
  Sum1 : Sum  Inputs=|+-
  Sum6 : Sum  Inputs=|+-
  Out1 : Outport
  wires:
  Gain2/1 -> Out1/1
  I/1 -> Sum/2
  Gain1/1 -> I/1
  Sum6/1 -> Gain1/1
  Sum1/1 -> Sum/1
  Sum/1 -> Gain2/1
  Gain/1 -> Sum1/1
  ref/1 -> Sum6/1, Gain/1
  y/1 -> Sum6/2, Sum1/2

== system lib_AC_GFM/GFM/VCC/dynamic/RC ==
  note: 1) Add Subsystem or Model blocks as valid variant choices.
      | 2) You cannot connect blocks at this level. At simulation, connectivity is automatically
      | determined, based on the active variant and port name matching.
  i_d_in : Inport
  i_d_out : Inport  Port=2
  i_q_in : Inport  Port=3
  i_q_out : Inport  Port=4
  omega : Inport  Port=5
  dynamic : Subsystem  VariantControl=rc_mode == 1
  static : Subsystem  VariantControl=rc_mode == 2
  static omega : Subsystem  VariantControl=(default)
  vd : Outport
  vq : Outport  Port=2

== system lib_AC_GFM/GFM/VCC/dynamic/RL ==
  note: 1) Add Subsystem or Model blocks as valid variant choices.
      | 2) You cannot connect blocks at this level. At simulation, connectivity is automatically
      | determined, based on the active variant and port name matching.
  v_in_d : Inport
  v_out_d : Inport  Port=2
  v_in_q : Inport  Port=3
  v_out_q : Inport  Port=4
  omega : Inport  Port=5
  dynamic : Subsystem  VariantControl=rl_mode == 1
      settings: PortSchema="{\"entries\":[{\"content\":{\"sides\":[{\"content\":{\"connectorIds\":[\"In1\"]},\"type\":\"ConnectorPlacement.EquallySpacedRectSide\",\"uuid\":\"63966e24-f9e7-4b2d-b456-7f4ea5e3f230\"},{\"content\":{\"connectorIds\":[\"In2\",\"In3\",\"In4\",\"In5\",\"Out1\",\"Out2\"],\"side\":\"RIGHT\"},\"type\":\"ConnectorPlacement.EquallySpacedRectSide\",\"uuid\":\"ded6ef04-52fd-47df-8e49-cf16b827098d\"},{\"content\":{\"side\":\"TOP\"},\"type\":\"ConnectorPlacement.EquallySpacedRectSide\",\"uuid\":\"f940a985-fa23-4968-ad44-1d76d0e20c6a\"}]},\"type\":\"ConnectorPlacement.EquallySpacedConnector\",\"uuid\":\"20f61d3c-9af2-4982-98ea-af4910e61c9c\"}],\"packageUris\":[\"http://schema.mathworks.com/mf0/Connector/R2020b\"],\"version\":\"1.0\"}"
  static : Subsystem  VariantControl=rl_mode == 2
  static_omega : Subsystem  VariantControl=(default)
  id : Outport
  iq : Outport  Port=2

== system lib_AC_GFM/GFM/VCC/dynamic/Subsystem ==
  In1 : Inport
  In2 : Inport  Port=2
  In3 : Inport  Port=3
  In4 : Inport  Port=4
  In5 : Inport  Port=5
  Constant : Constant  Value=Tint==Inf  VectorParams1D=off
  Switch{,1..4} (5 alike) : Switch  Criteria=u2 > Threshold  SaturateOnIntegerOverflow=off  InputSameDT=off
  Zero : Constant  Value=0  OutDataTypeStr=Inherit: Inherit via back propagation
  Out1 : Outport
  Out2 : Outport  Port=2
  Out3 : Outport  Port=3
  Out4 : Outport  Port=4
  Out5 : Outport  Port=5
  wires:
  Zero/1 -> Switch/1
  In1/1 -> Switch4/1, Switch3/1, Switch2/1, Switch1/1, Switch/3
  Switch/1 -> Out1/1
  Constant/1 -> Switch/2, Switch4/2, Switch3/2, Switch2/2, Switch1/2
  Switch1/1 -> Out2/1
  Switch2/1 -> Out3/1
  Switch3/1 -> Out4/1
  In3/1 -> Switch2/3
  In4/1 -> Switch3/3
  In2/1 -> Switch1/3
  Switch4/1 -> Out5/1
  In5/1 -> Switch4/3

== system lib_AC_GFM/GFM/VCC/dynamic/Subsystem1 ==
  id : Inport
  iod : Inport  Port=2
  iq : Inport  Port=3
  ioq : Inport  Port=4
  In5 : Inport  Port=5
  Constant : Constant  Value=Text==Inf  VectorParams1D=off
  Switch{,1..4} (5 alike) : Switch  Criteria=u2 > Threshold  SaturateOnIntegerOverflow=off  InputSameDT=off
  Zero : Constant  Value=0  OutDataTypeStr=Inherit: Inherit via back propagation
  Out1 : Outport
  Out2 : Outport  Port=2
  Out3 : Outport  Port=3
  Out4 : Outport  Port=4
  Out5 : Outport  Port=5
  wires:
  In5/1 -> Switch4/3
  Switch4/1 -> Out5/1
  iod/1 -> Switch1/3
  ioq/1 -> Switch3/3
  iq/1 -> Switch2/3
  Switch3/1 -> Out4/1
  Switch2/1 -> Out3/1
  Switch1/1 -> Out2/1
  Constant/1 -> Switch1/2, Switch2/2, Switch3/2, Switch4/2, Switch/2
  Switch/1 -> Out1/1
  id/1 -> Switch/3, Switch1/1, Switch2/1, Switch3/1, Switch4/1
  Zero/1 -> Switch/1

== system lib_AC_GFM/GFM/VCC/dynamic_VC/RC ==
  note: 1) Add Subsystem or Model blocks as valid variant choices.
      | 2) You cannot connect blocks at this level. At simulation, connectivity is automatically
      | determined, based on the active variant and port name matching.
  i_d_in : Inport
  i_d_out : Inport  Port=2
  i_q_in : Inport  Port=3
  i_q_out : Inport  Port=4
  omega : Inport  Port=5
  dynamic : Subsystem  VariantControl=rc_mode == 1
  static : Subsystem  VariantControl=rc_mode == 2
  static omega : Subsystem  VariantControl=(default)
  vd : Outport
  vq : Outport  Port=2

== system lib_AC_GFM/GFM/VCC/dynamic_VC/Subsystem ==
  ref : Inport
  y : Inport  Port=2
  Gain : Gain  Gain=Bext
  Gain1 : Gain  Gain=1./Text
  Gain2 : Gain  Gain=Kext
  Integrator : Integrator  InitialCondition=op_GFM.VCC_dynamic_VC_Subsystem_Integrator
  Sum : Sum  Inputs=++|
  Sum1 : Sum  Inputs=|+-
  Sum6 : Sum  Inputs=|+-
  Out1 : Outport
  wires:
  y/1 -> Sum1/2, Sum6/2
  ref/1 -> Gain/1, Sum6/1
  Gain/1 -> Sum1/1
  Sum/1 -> Gain2/1
  Sum1/1 -> Sum/1
  Sum6/1 -> Gain1/1
  Gain1/1 -> Integrator/1
  Integrator/1 -> Sum/2
  Gain2/1 -> Out1/1

== system lib_AC_GFM/GFM/VCC/dynamic_VC/Subsystem1 ==
  ref : Inport
  y : Inport  Port=2
  Gain : Gain  Gain=Bext
  Gain1 : Gain  Gain=1./Text
  Gain2 : Gain  Gain=Kext
  Integrator : Integrator  InitialCondition=op_GFM.VCC_dynamic_VC_Subsystem1_Integrator
  Sum : Sum  Inputs=++|
  Sum1 : Sum  Inputs=|+-
  Sum6 : Sum  Inputs=|+-
  Out1 : Outport
  wires:
  Gain2/1 -> Out1/1
  Integrator/1 -> Sum/2
  Gain1/1 -> Integrator/1
  Sum6/1 -> Gain1/1
  Sum1/1 -> Sum/1
  Sum/1 -> Gain2/1
  Gain/1 -> Sum1/1
  ref/1 -> Sum6/1, Gain/1
  y/1 -> Sum6/2, Sum1/2

== system lib_AC_GFM/GFM/VCC/dynamic_limiting/PIid ==
  ref : Inport
  y : Inport  Port=2
  Gain : Gain  Gain=Bint
  Gain1 : Gain  Gain=1./Tint
  Gain2 : Gain  Gain=Kint
  I : Integrator  InitialCondition=op_GFM.VCC_dynamic_limiting_PIid_I
  Sum : Sum  Inputs=++|
  Sum1 : Sum  Inputs=|+-
  Sum6 : Sum  Inputs=|+-
  Out1 : Outport
  wires:
  y/1 -> Sum1/2, Sum6/2
  ref/1 -> Gain/1, Sum6/1
  Gain/1 -> Sum1/1
  Sum/1 -> Gain2/1
  Sum1/1 -> Sum/1
  Sum6/1 -> Gain1/1
  Gain1/1 -> I/1
  I/1 -> Sum/2
  Gain2/1 -> Out1/1

== system lib_AC_GFM/GFM/VCC/dynamic_limiting/PIiq ==
  ref : Inport
  y : Inport  Port=2
  Gain : Gain  Gain=Bint
  Gain1 : Gain  Gain=1./Tint
  Gain2 : Gain  Gain=Kint
  I : Integrator  InitialCondition=op_GFM.VCC_dynamic_limiting_PIiq_I
  Sum : Sum  Inputs=++|
  Sum1 : Sum  Inputs=|+-
  Sum6 : Sum  Inputs=|+-
  Out1 : Outport
  wires:
  Gain2/1 -> Out1/1
  I/1 -> Sum/2
  Gain1/1 -> I/1
  Sum6/1 -> Gain1/1
  Sum1/1 -> Sum/1
  Sum/1 -> Gain2/1
  Gain/1 -> Sum1/1
  ref/1 -> Sum6/1, Gain/1
  y/1 -> Sum6/2, Sum1/2
